simulink model "Drive_DC"  (R2022b)
settings: Solver=VariableStepAuto  StartTime=0.0  StopTime=13  MaxStep=1e-5  RelTol=1e-3
undefined symbols (not defined in the file or in its folder): DiscIntNeverNeededParam, sigbuilder_block
libraries: spsMeanLib x6, slpidlib x5, simulink_extras x5, spsSawtoothGeneratorLib x4, simulink x2, pid_lib x1, spspowerguiLib x1
(part 1 of 2)
settings Model: Creator=AHMED  LastModifiedBy=moham
settings SolverCC: ZeroCrossAlgorithm=Adaptive
settings DebuggingCC: MaskedZcDiagnostic=none  IgnoredZcDiagnostic=none  UnconnectedInputMsg=warning  UnconnectedOutputMsg=warning  UnconnectedLineMsg=warning
settings ModelReferenceCC: EnableRefExpFcnMdlSchedulingChecks=on
settings RTWCC: DLArmComputeVersion=19.05

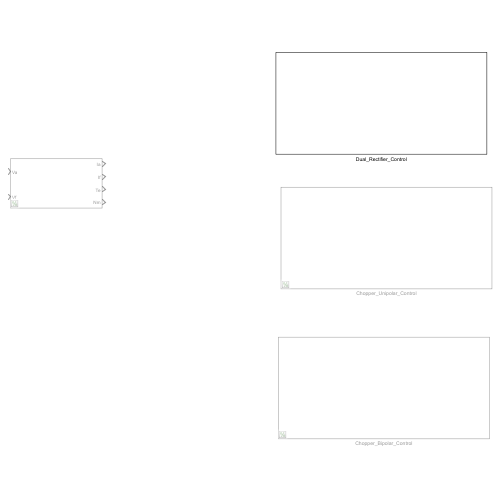
[thumbnail: Simulink's stored preview of the top-level diagram]
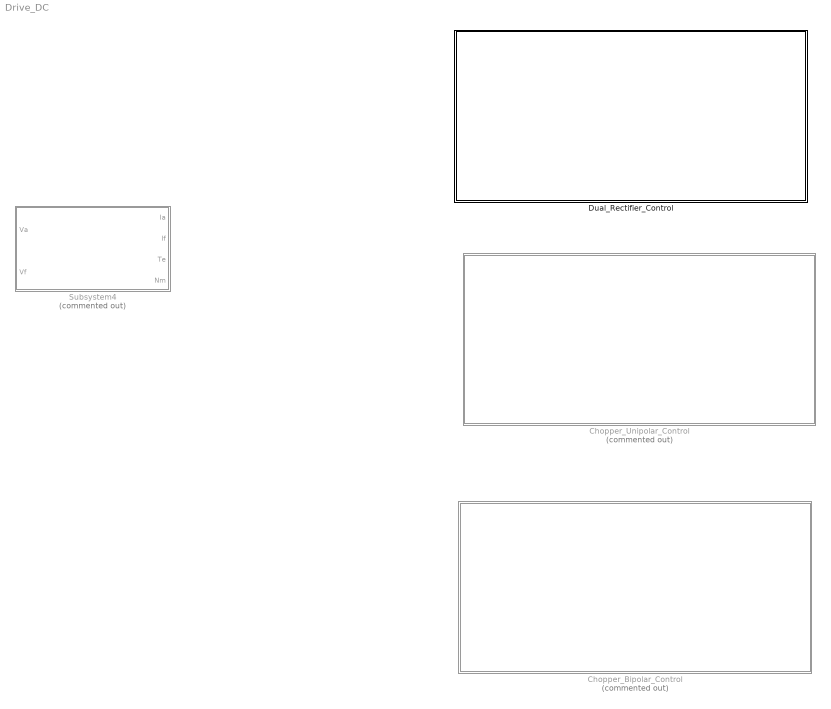
== system Drive_DC ==
  Chopper_Bipolar_Control : Subsystem  Commented=on
  Chopper_Unipolar_Control : Subsystem  Commented=on
  Dual_Rectifier_Control : Subsystem
  Subsystem4 : Subsystem  Commented=on  mask{Ra=0.6, Rf=240, La=12e-3, Lf=120, J=0.1, k=1.309}

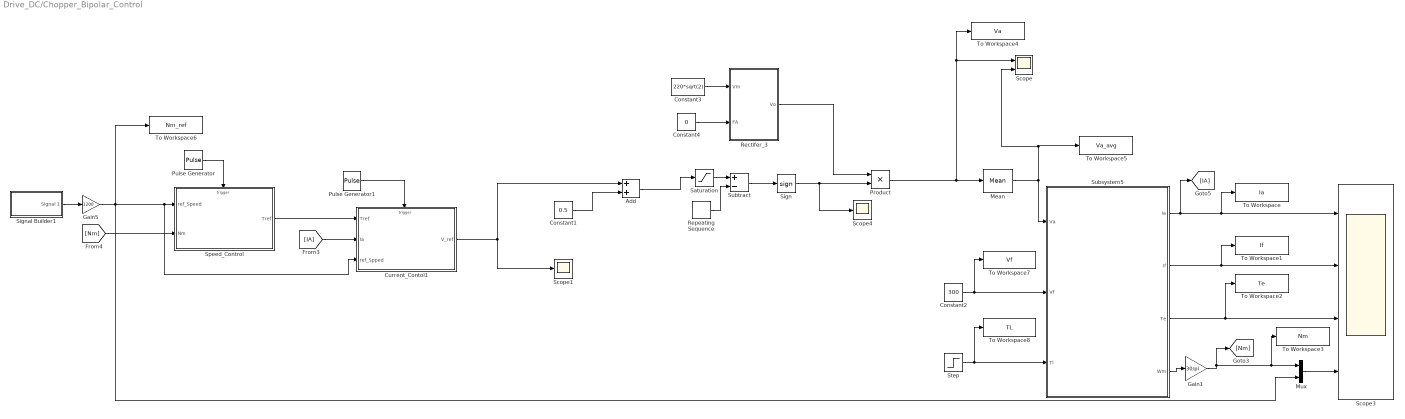
== system Drive_DC/Chopper_Bipolar_Control ==
  Add : Sum
  Constant1 : Constant  Value=0.5
  Constant2 : Constant  Value=300
  Constant3 : Constant  Value=220*sqrt(2)
  Constant4 : Constant  Value=0
  Current_Contol1 : Subsystem
  Gain1 : Gain  Gain=30/pi
  Gain5 : Gain  Gain=1200
  Mean : spsMeanLib/Mean  Freq=50  Vinit=0  Ts=0
  Mux : Mux  Inputs=2
  Product : Product
  Pulse Generator : DiscretePulseGenerator  PulseType=Time based  Period=1/1000  PulseWidth=50
  Pulse Generator1 : DiscretePulseGenerator  PulseType=Time based  Period=1/10000  PulseWidth=50
  Rectifer_3 : Subsystem
  Repeating Sequence : simulink/Sources/Repeating Sequence  rep_seq_t=[0 0.5/10000 1/10000]  rep_seq_y=[0 1 0]
  Saturation : Saturate  UpperLimit=1  LowerLimit=0
  Scope : Scope  NumInputPorts=2
  Scope1 : Scope
  Scope3 : Scope  NumInputPorts=4
  Scope4 : Scope
  Sign : Signum
  Signal Builder1 : Subsystem  Tag=STV Subsys  LoadFcn=sigbuilder_block('load');  StartFcn=sigbuilder_block('start');  StopFcn=sigbuilder_block('stop');  ClipboardFcn=sigbuilder_block('clipboard');  mask(Sigbuilder block){tuvar=[0:10]}
      mask help: Simulink:masks:SigbuilderBlock_MD
      mask init:
      | if ~strcmp(get_param(bdroot(gcbh),'SimulationStatus'),'stopped') tuvar = sigbuilder_block('maskInit'); end
      settings: CopyFcn=sigbuilder_block('copy');  DeleteFcn=sigbuilder_block('delete');  ModelCloseFcn=sigbuilder_block('modelClose');  PreSaveFcn=sigbuilder_block('preSave');  PauseFcn=sigbuilder_block('pause');  ContinueFcn=sigbuilder_block('continue');  NameChangeFcn=sigbuilder_block('namechange');  OpenFcn=sigbuilder_block('open',[5.4 30 1141.2 522.6 ]);  CloseFcn=sigbuilder_block('close');
      mask Display: plot(0, 0, 100, 100,[2, 2, 32, 32, 2], [68, 8, 8, 68, 68],[32, 2], [38, 38], [32, 19, 2],[53, 60, 44], [32, 17, 17, 2],[16, 16, 31, 31]);txt = getActiveGroup(gcbh);text(2, 100, txt,'verticalAlignment', 'top');
  Speed_Control : Subsystem
  Step : Step  Time=2.25  After=5  SampleTime=0
  Subsystem5 : Subsystem  mask{Ra=0.6, Rf=240, La=12e-3, Lf=120, J=0.05, k=1.309}
  Subtract : Sum  Inputs=+-
  To Workspace : ToWorkspace  VariableName=Ia  SaveFormat=Structure With Time  SampleTime=-1
  To Workspace1 : ToWorkspace  VariableName=If  SaveFormat=Structure With Time  SampleTime=-1
  To Workspace2 : ToWorkspace  VariableName=Te  SaveFormat=Structure With Time  SampleTime=-1
  To Workspace3 : ToWorkspace  VariableName=Nm  SaveFormat=Structure With Time  SampleTime=-1
  To Workspace4 : ToWorkspace  VariableName=Va  SaveFormat=Structure With Time  SampleTime=-1
  To Workspace5 : ToWorkspace  VariableName=Va_avg  SaveFormat=Structure With Time  SampleTime=-1
  To Workspace6 : ToWorkspace  VariableName=Nm_ref  SaveFormat=Structure With Time  SampleTime=-1
  To Workspace7 : ToWorkspace  VariableName=Vf  SaveFormat=Structure With Time  SampleTime=-1
  To Workspace8 : ToWorkspace  VariableName=TL  SaveFormat=Structure With Time  SampleTime=-1
  wires:
  Subtract/1 -> Sign/1
  Mean/1 -> Subsystem5/1(Va), To Workspace5/1, Scope/2
  Rectifer_3/1(Vo) -> Product/1
  Sign/1 -> Scope4/1, Product/2
  Current_Contol1/1(V_ref) -> Add/1, Scope1/1
  Repeating Sequence/1 -> Subtract/2
  Gain1/1 -> Mux/1, To Workspace3/1, [Nm]
  Subsystem5/2(If) -> Scope3/2, To Workspace1/1
  Mux/1 -> Scope3/4
  Step/1 -> To Workspace8/1, Subsystem5/3(Tl)
  Speed_Control/1(Tref) -> Current_Contol1/1(Tref)
  Constant2/1 -> To Workspace7/1, Subsystem5/2(Vf)
  Product/1 -> To Workspace4/1, Scope/1, Mean/1
  [IA] -> Current_Contol1/2(Ia)
  Subsystem5/4(Wm) -> Gain1/1
  Signal Builder1/1(Signal 1) -> Gain5/1
  Gain5/1 -> To Workspace6/1, Mux/2, Current_Contol1/3("ref_Spped "), Speed_Control/1(ref_Speed)
  [Nm] -> Speed_Control/2("Nm ")
  Pulse Generator/1 -> Speed_Control/Trigger
  Subsystem5/3(Te) -> Scope3/3, To Workspace2/1
  Pulse Generator1/1 -> Current_Contol1/Trigger
  Subsystem5/1(Ia) -> [IA], Scope3/1, To Workspace/1
  Constant1/1 -> Add/2
  Add/1 -> Saturation/1
  Saturation/1 -> Subtract/1
  Constant3/1 -> Rectifer_3/1(Vm)
  Constant4/1 -> Rectifer_3/2(FA)

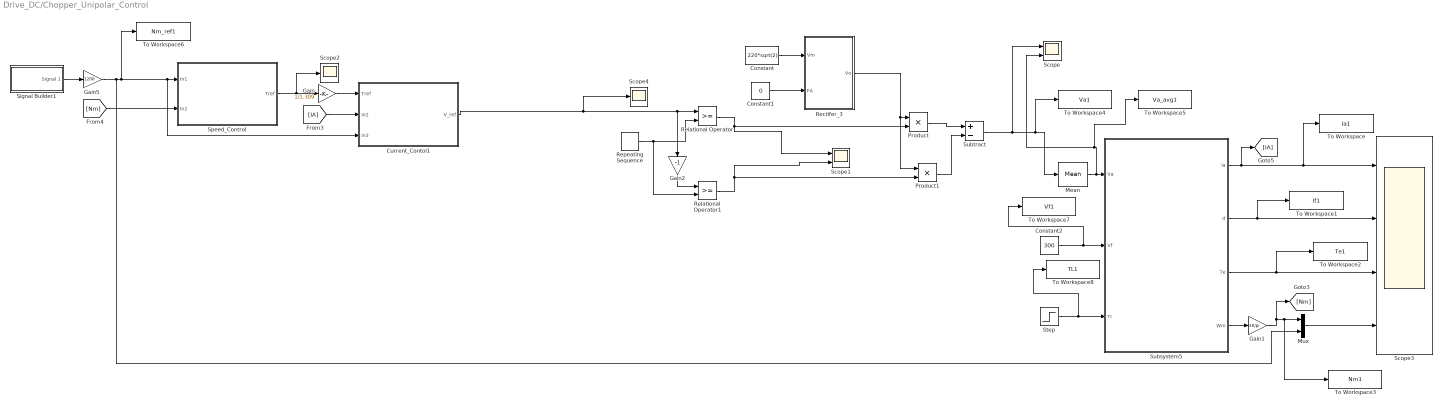
== system Drive_DC/Chopper_Unipolar_Control ==
  Constant : Constant  Value=220*sqrt(2)
  Constant1 : Constant  Value=0
  Constant2 : Constant  Value=300
  Current_Contol1 : Subsystem
  Gain : Gain  Gain=1/1.309
  Gain1 : Gain  Gain=30/pi
  Gain2 : Gain  Gain=-1
  Gain5 : Gain  Gain=1200
  Mean : spsMeanLib/Mean  Freq=50  Vinit=0  Ts=0
  Mux : Mux  Inputs=2
  Product : Product
  Product1 : Product
  Rectifer_3 : Subsystem
  Relational Operator : RelationalOperator  OutDataTypeStr=boolean  RndMeth=Simplest  InputSameDT=off
  Relational Operator1 : RelationalOperator  OutDataTypeStr=boolean  RndMeth=Simplest  InputSameDT=off
  Repeating Sequence : simulink/Sources/Repeating Sequence  rep_seq_t=[0 0.5/1000 1/1000]  rep_seq_y=[0 1 0]
  Scope : Scope  NumInputPorts=2
  Scope1 : Scope  NumInputPorts=2
  Scope2 : Scope
  Scope3 : Scope  NumInputPorts=4
  Scope4 : Scope
  Signal Builder1 : Subsystem  Tag=STV Subsys  LoadFcn=sigbuilder_block('load');  StartFcn=sigbuilder_block('start');  StopFcn=sigbuilder_block('stop');  ClipboardFcn=sigbuilder_block('clipboard');  mask(Sigbuilder block){tuvar=[0:10]}
      mask help: Simulink:masks:SigbuilderBlock_MD
      mask init:
      | if ~strcmp(get_param(bdroot(gcbh),'SimulationStatus'),'stopped') tuvar = sigbuilder_block('maskInit'); end
      settings: CopyFcn=sigbuilder_block('copy');  DeleteFcn=sigbuilder_block('delete');  ModelCloseFcn=sigbuilder_block('modelClose');  PreSaveFcn=sigbuilder_block('preSave');  PauseFcn=sigbuilder_block('pause');  ContinueFcn=sigbuilder_block('continue');  NameChangeFcn=sigbuilder_block('namechange');  OpenFcn=sigbuilder_block('open',[5.4 30 1141.2 522.6 ]);  CloseFcn=sigbuilder_block('close');
      mask Display: plot(0, 0, 100, 100,[2, 2, 32, 32, 2], [68, 8, 8, 68, 68],[32, 2], [38, 38], [32, 19, 2],[53, 60, 44], [32, 17, 17, 2],[16, 16, 31, 31]);txt = getActiveGroup(gcbh);text(2, 100, txt,'verticalAlignment', 'top');
  Speed_Control : Subsystem
  Step : Step  Time=2.25  After=5  SampleTime=0
  Subsystem5 : Subsystem  mask{Ra=0.6, Rf=240, La=12e-3, Lf=120, J=0.05, k=1.309}
  Subtract : Sum  Inputs=+-
  To Workspace : ToWorkspace  VariableName=Ia1  SaveFormat=Structure With Time  SampleTime=-1
  To Workspace1 : ToWorkspace  VariableName=If1  SaveFormat=Structure With Time  SampleTime=-1
  To Workspace2 : ToWorkspace  VariableName=Te1  SaveFormat=Structure With Time  SampleTime=-1
  To Workspace3 : ToWorkspace  VariableName=Nm1  SaveFormat=Structure With Time  SampleTime=-1
  To Workspace4 : ToWorkspace  VariableName=Va1  SaveFormat=Structure With Time  SampleTime=-1
  To Workspace5 : ToWorkspace  VariableName=Va_avg1  SaveFormat=Structure With Time  SampleTime=-1
  To Workspace6 : ToWorkspace  VariableName=Nm_ref1  SaveFormat=Structure With Time  SampleTime=-1
  To Workspace7 : ToWorkspace  VariableName=Vf1  SaveFormat=Structure With Time  SampleTime=-1
  To Workspace8 : ToWorkspace  VariableName=TL1  SaveFormat=Structure With Time  SampleTime=-1
  wires:
  Subsystem5/3(Te) -> To Workspace2/1, Scope3/3
  [Nm] -> Speed_Control/2(In2)
  Gain5/1 -> To Workspace6/1, Speed_Control/1(In1), Current_Contol1/3(In3), Mux/2
  Signal Builder1/1(Signal 1) -> Gain5/1
  Subsystem5/4(Wm) -> Gain1/1
  [IA] -> Current_Contol1/2(In2)
  Subtract/1 -> Scope/1, To Workspace4/1, Mean/1
  Constant2/1 -> To Workspace7/1, Subsystem5/2(Vf)
  Speed_Control/1(Tref) -> Scope2/1, Gain/1
  Step/1 -> To Workspace8/1, Subsystem5/3(Tl)
  Mux/1 -> Scope3/4
  Subsystem5/1(Ia) -> To Workspace/1, Scope3/1, [IA]
  Subsystem5/2(If) -> To Workspace1/1, Scope3/2
  Gain1/1 -> [Nm], To Workspace3/1, Mux/1
  Repeating Sequence/1 -> Relational Operator1/2, Relational Operator/2
  Current_Contol1/1(V_ref) -> Scope4/1, Relational Operator/1, Gain2/1
  Rectifer_3/1(Vo) -> Product1/1, Product/1
  Product/1 -> Subtract/1
  Product1/1 -> Subtract/2
  Mean/1 -> To Workspace5/1, Scope/2, Subsystem5/1(Va)
  Relational Operator/1 -> Product/2, Scope1/1
  Relational Operator1/1 -> Product1/2, Scope1/2
  Gain2/1 -> Relational Operator1/1
  Constant/1 -> Rectifer_3/1(Vm)
  Constant1/1 -> Rectifer_3/2(FA)
  Gain/1 -> Current_Contol1/1(Tref)

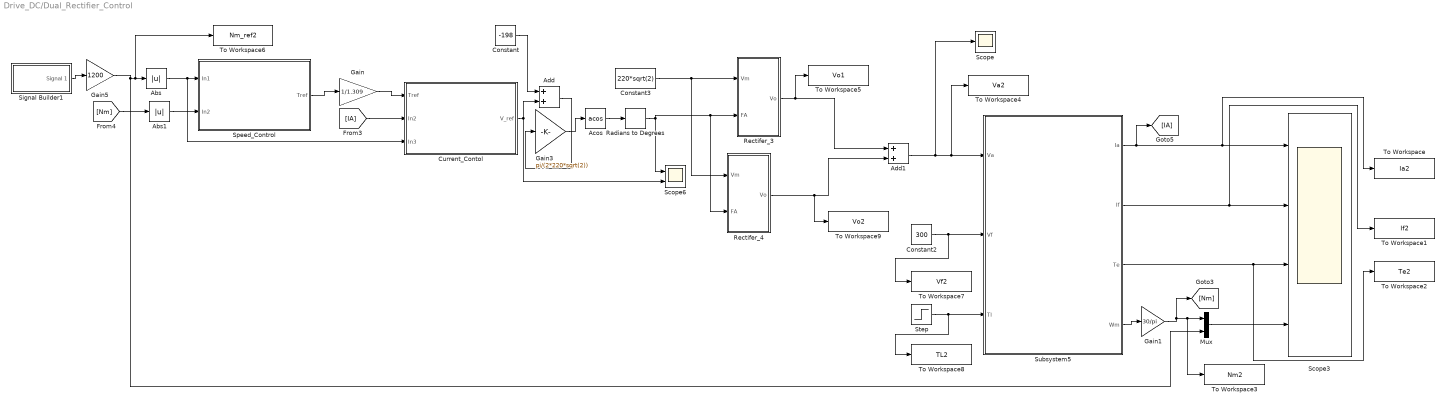
== system Drive_DC/Dual_Rectifier_Control ==
  Abs : Abs  SaturateOnIntegerOverflow=off
  Abs1 : Abs  SaturateOnIntegerOverflow=off
  Acos : Trigonometry  Operator=acos
  Add : Sum
  Add1 : Sum
  Constant : Constant  Value=-198
  Constant2 : Constant  Value=300
  Constant3 : Constant  Value=220*sqrt(2)
  Current_Contol : Subsystem
  Gain : Gain  Gain=1/1.309
  Gain1 : Gain  Gain=30/pi
  Gain3 : Gain  Gain=pi/(2*220*sqrt(2))
  Gain5 : Gain  Gain=1200
  Mux : Mux  Inputs=2
  Radians to Degrees : simulink_extras/Transformations/Radians to Degrees
  Rectifer_3 : Subsystem
  Rectifer_4 : Subsystem
  Scope : Scope
  Scope3 : Scope  NumInputPorts=4
  Scope6 : Scope  NumInputPorts=2
  Signal Builder1 : Subsystem  Tag=STV Subsys  LoadFcn=sigbuilder_block('load');  StartFcn=sigbuilder_block('start');  StopFcn=sigbuilder_block('stop');  ClipboardFcn=sigbuilder_block('clipboard');  mask(Sigbuilder block){tuvar=[0:10]}
      mask help: Simulink:masks:SigbuilderBlock_MD
      mask init:
      | if ~strcmp(get_param(bdroot(gcbh),'SimulationStatus'),'stopped') tuvar = sigbuilder_block('maskInit'); end
      settings: CopyFcn=sigbuilder_block('copy');  DeleteFcn=sigbuilder_block('delete');  ModelCloseFcn=sigbuilder_block('modelClose');  PreSaveFcn=sigbuilder_block('preSave');  PauseFcn=sigbuilder_block('pause');  ContinueFcn=sigbuilder_block('continue');  NameChangeFcn=sigbuilder_block('namechange');  OpenFcn=sigbuilder_block('open',[5.4 30 1141.2 522.6 ]);  CloseFcn=sigbuilder_block('close');
      mask Display: plot(0, 0, 100, 100,[2, 2, 32, 32, 2], [68, 8, 8, 68, 68],[32, 2], [38, 38], [32, 19, 2],[53, 60, 44], [32, 17, 17, 2],[16, 16, 31, 31]);txt = getActiveGroup(gcbh);text(2, 100, txt,'verticalAlignment', 'top');
  Speed_Control : Subsystem
  Step : Step  Time=2.25  After=5  SampleTime=0
  Subsystem5 : Subsystem  mask{Ra=0.6, Rf=240, La=12e-3, Lf=120, J=0.05, k=1.309}
  To Workspace : ToWorkspace  VariableName=Ia2  SaveFormat=Structure With Time  SampleTime=-1
  To Workspace1 : ToWorkspace  VariableName=If2  SaveFormat=Structure With Time  SampleTime=-1
  To Workspace2 : ToWorkspace  VariableName=Te2  SaveFormat=Structure With Time  SampleTime=-1
  To Workspace3 : ToWorkspace  VariableName=Nm2  SaveFormat=Structure With Time  SampleTime=-1
  To Workspace4 : ToWorkspace  VariableName=Va2  SaveFormat=Structure With Time  SampleTime=-1
  To Workspace5 : ToWorkspace  VariableName=Vo1  SaveFormat=Structure With Time  SampleTime=-1
  To Workspace6 : ToWorkspace  VariableName=Nm_ref2  SaveFormat=Structure With Time  SampleTime=-1
  To Workspace7 : ToWorkspace  VariableName=Vf2  SaveFormat=Structure With Time  SampleTime=-1
  To Workspace8 : ToWorkspace  VariableName=TL2  SaveFormat=Structure With Time  SampleTime=-1
  To Workspace9 : ToWorkspace  VariableName=Vo2  SaveFormat=Structure With Time  SampleTime=-1
  wires:
  [Nm] -> Abs1/1
  Gain1/1 -> To Workspace3/1, Mux/1, [Nm]
  Gain5/1 -> Mux/2, To Workspace6/1, Abs/1
  Subsystem5/2(If) -> To Workspace1/1, Scope3/2
  Subsystem5/1(Ia) -> [IA], To Workspace/1, Scope3/1
  Mux/1 -> Scope3/4
  Step/1 -> To Workspace8/1, Subsystem5/3(Tl)
  Gain3/1 -> Acos/1
  Speed_Control/1(Tref) -> Gain/1
  Constant2/1 -> To Workspace7/1, Subsystem5/2(Vf)
  Acos/1 -> Radians to Degrees/1
  Add1/1 -> Scope/1, To Workspace4/1, Subsystem5/1(Va)
  Radians to Degrees/1 -> Rectifer_4/2(FA), Rectifer_3/2(FA), Scope6/1
  [IA] -> Current_Contol/2(In2)
  Subsystem5/4(Wm) -> Gain1/1
  Signal Builder1/1(Signal 1) -> Gain5/1
  Abs/1 -> Current_Contol/3(In3), Speed_Control/1(In1)
  Abs1/1 -> Speed_Control/2(In2)
  Constant3/1 -> Rectifer_3/1(Vm), Rectifer_4/1(Vm)
  Current_Contol/1(V_ref) -> Add/2, Scope6/2
  Subsystem5/3(Te) -> To Workspace2/1, Scope3/3
  Add/1 -> Gain3/1
  Constant/1 -> Add/1
  Gain/1 -> Current_Contol/1(Tref)
  Rectifer_3/1(Vo) -> To Workspace5/1, Add1/1
  Rectifer_4/1(Vo) -> To Workspace9/1, Add1/2

== system Drive_DC/Subsystem4 ==
  Va : Inport
  Vf : Inport  Port=2
  Constant : Constant  Value=1000
  Gain : Gain  Gain=pi/30
  Subsystem : Subsystem
  Subsystem1 : Subsystem
  Subsystem3 : Subsystem
  Ia : Outport
  If : Outport  Port=2
  Te : Outport  Port=3
  Nm : Outport  Port=4
  wires:
  Va/1 -> Subsystem/1(Va)
  Subsystem/1(Ia) -> Subsystem1/1(Ia), Ia/1
  Subsystem1/1(Te) -> Te/1
  Vf/1 -> Subsystem3/1(In1)
  Subsystem3/1(Out1) -> If/1
  Constant/1 -> Gain/1
  Gain/1 -> Nm/1, Subsystem/2(W)

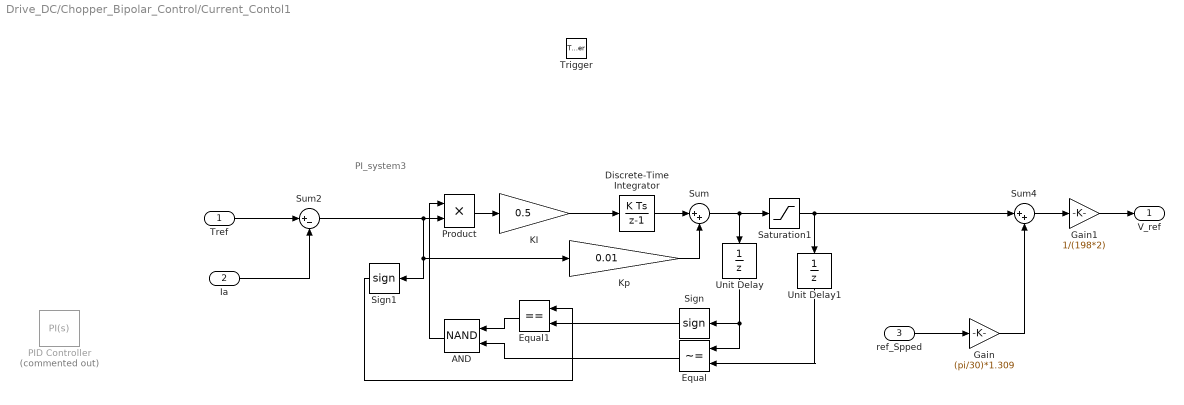
== system Drive_DC/Chopper_Bipolar_Control/Current_Contol1 ==
  note: PI_system3
  Tref : Inport
  Ia : Inport  Port=2
  "ref_Spped " : Inport  Port=3
  Trigger : TriggerPort  VariantControl=(inherit)  PortDimensions=1
  AND : Logic  Operator=NAND  AllPortsSameDT=off  OutDataTypeStr=boolean
  Discrete-Time Integrator : DiscreteIntegrator  SampleTime=-1  ICPrevOutput=DiscIntNeverNeededParam  ICPrevScaledInput=DiscIntNeverNeededParam
  Equal : RelationalOperator  Operator=~=  OutDataTypeStr=boolean  RndMeth=Simplest  InputSameDT=off
  Equal1 : RelationalOperator  Operator===  OutDataTypeStr=boolean  RndMeth=Simplest  InputSameDT=off
  Gain : Gain  Gain=(pi/30)*1.309
  Gain1 : Gain  Gain=1/(198*2)
  KI : Gain  Gain=0.5
  Kp : Gain  Gain=0.01
  PID Controller : slpidlib/PID Controller  Commented=on  Controller=PI  Form=Parallel  TimeDomain=Continuous-time  UseExternalTs=off  SampleTime=-1  IntegratorMethod=Forward Euler  FilterMethod=Forward Euler  ControllerParametersSource=internal  P=0.1  I=10  UseKiTs=off  D=0  N=100  UseFilter=on  TunerSelectOption=Transfer Function Based (PID Tuner App)  InitialConditionSource=internal  InitialConditionForIntegrator=0  InitialConditionForFilter=0  DifferentiatorICPrevScaledInput=0  ExternalReset=none  TrackingMode=off  Kt=1  LimitOutput=on  SatLimitsSource=internal  UpperSaturationLimit=240  LowerSaturationLimit=-240  LinearizeAsGain=on  AntiWindupMode=clamping  Kb=1  LimitIntegrator=off  UpperIntegratorSaturationLimit=inf  LowerIntegratorSaturationLimit=-inf  POutMin=[]  POutMax=[]  IOutMin=[]  IOutMax=[]  DOutMin=[]  DOutMax=[]  NOutMin=[]  NOutMax=[]  SumOutMin=[]  SumOutMax=[]  SaturationOutMin=[]  SaturationOutMax=[]  PParamMin=[]  PParamMax=[]  IParamMin=[]  IParamMax=[]  DParamMin=[]  DParamMax=[]  NParamMin=[]  NParamMax=[]  KbParamMin=[]  KbParamMax=[]  KtParamMin=[]  KtParamMax=[]  KbOutMin=[]  KbOutMax=[]  KtOutMin=[]  KtOutMax=[]  IntegratorOutMin=[]  IntegratorOutMax=[]  FilterOutMin=[]  FilterOutMax=[]  SumI1OutMin=[]  SumI1OutMax=[]  SumI2OutMin=[]  SumI2OutMax=[]  SumI3OutMin=[]  SumI3OutMax=[]  SumI4OutMin=[]  SumI4OutMax=[]  SumDOutMin=[]  SumDOutMax=[]  DifferentiatorOutMin=[]  DifferentiatorOutMax=[]  FilterDiffOutCoefMin=[]  FilterDiffOutCoefMax=[]  ReciprocalOutMin=[]  ReciprocalOutMax=[]  SumDenOutMin=[]  SumDenOutMax=[]  SumNumOutMin=[]  SumNumOutMax=[]  DivideOutMin=[]  DivideOutMax=[]  UdiffTsProdOutMin=[]  UdiffTsProdOutMax=[]  NTsProdOutMin=[]  NTsProdOutMax=[]  UintegralTsProdOutMin=[]  UintegralTsProdOutMax=[]  UngainTsProdOutMin=[]  UngainTsProdOutMax=[]  ClampingZeroOutDataTypeStr=Inherit: Inherit via back propagation  ClampingZeroOutMin=[]  ClampingZeroOutMax=[]  FilterDenConstantOutDataTypeStr=Inherit: Inherit via back propagation  FilterDenConstantOutMin=[]  FilterDenConstantOutMax=[]  PCopyOutDataTypeStr=Inherit: Inherit via back propagation  PCopyOutMin=[]  PCopyOutMax=[]  NCopyOutDataTypeStr=Inherit: Inherit via back propagation  NCopyOutMin=[]  NCopyOutMax=[]  IntegratorContinuousStateAttributes=''  IntegratorStateMustResolveToSignalObject=off  IntegratorRTWStateStorageClass=Auto  FilterContinuousStateAttributes=''  FilterStateMustResolveToSignalObject=off  FilterRTWStateStorageClass=Auto  ParallelPVariant=InternalParameters  IdealPVariant=Disabled  IVariant=InternalParameters  DVariant=Disabled  IntegratorVariant=Continuous  SatVariant=Enabled  AWVariant=ContClampingParallel  PCopyVariant=Disabled  TRVariant=Disabled  FdbkBlocksVariant=Forward  IdealPFdbkVariant=Disabled  SatFdbkVariant=Disabled  DerivativeFilterVariant=Disabled  NVariant=Disabled  NCopyVariant=Disabled_SignalSpec  FilterICVariant=Disabled  IntegratorICVariant=InternalICs  ExternalResetVariant=Disabled  TRSumVariant=Passthrough  SumFdbkVariant=Disabled  SumVariant=Sum_PI  TsampFilterVariant=InternalTs  TsampNgainVariant=Passthrough  TsampIntegralVariant=Passthrough  ExternalSaturationOutDataTypeStr=Inherit: Same as second input
  Product : Product
  Saturation1 : Saturate  UpperLimit=198*2  LowerLimit=0
  Sign : Signum
  Sign1 : Signum
  Sum : Sum  Inputs=|++
  Sum2 : Sum  Inputs=|+-
  Sum4 : Sum  Inputs=|++
  Unit Delay : UnitDelay  SampleTime=-1  HasFrameUpgradeWarning=on
  Unit Delay1 : UnitDelay  SampleTime=-1  HasFrameUpgradeWarning=on
  V_ref : Outport
  wires:
  Gain1/1 -> V_ref/1
  Tref/1 -> Sum2/1
  Ia/1 -> Sum2/2
  "ref_Spped "/1 -> Gain/1
  Gain/1 -> Sum4/2
  Discrete-Time Integrator/1 -> Sum/1
  Kp/1 -> Sum/2
  KI/1 -> Discrete-Time Integrator/1
  Sum/1 -> Saturation1/1, Unit Delay/1
  Saturation1/1 -> Sum4/1, Unit Delay1/1
  Sign/1 -> Equal1/2
  Sign1/1 -> Equal1/1
  Equal1/1 -> AND/1
  Equal/1 -> AND/2
  Unit Delay/1 -> Equal/1, Sign/1
  Product/1 -> KI/1
  Unit Delay1/1 -> Equal/2
  AND/1 -> Product/1
  Sum2/1 -> Kp/1, Sign1/1, Product/2
  Sum4/1 -> Gain1/1

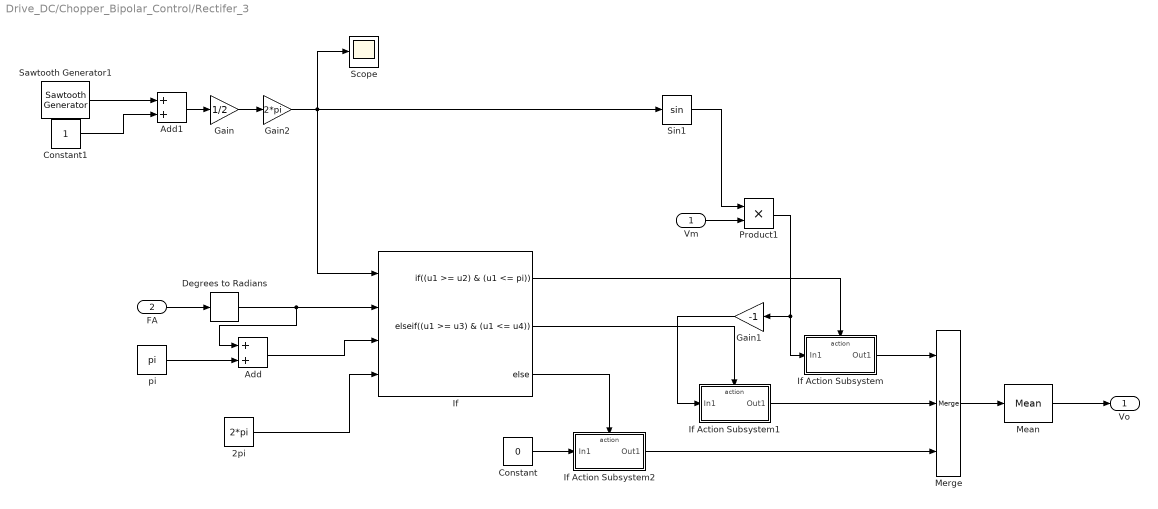
== system Drive_DC/Chopper_Bipolar_Control/Rectifer_3 ==
  Vm : Inport
  FA : Inport  Port=2
  2pi : Constant  Value=2*pi
  Add : Sum
  Add1 : Sum
  Constant : Constant  Value=0
  Constant1 : Constant
  Degrees to Radians : simulink_extras/Transformations/Degrees to Radians
  Gain : Gain  Gain=1/2
  Gain1 : Gain  Gain=-1
  Gain2 : Gain  Gain=2*pi
  If : If  NumInputs=4  IfExpression=(u1 >= u2) & (u1 <= pi)  ElseIfExpressions=(u1 >= u3) & (u1 <= u4)
  If Action Subsystem : Subsystem  TreatAsAtomicUnit=on
  If Action Subsystem1 : Subsystem  TreatAsAtomicUnit=on
  If Action Subsystem2 : Subsystem  TreatAsAtomicUnit=on
  Mean : spsMeanLib/Mean  Freq=50  Vinit=0  Ts=0
  Merge : Merge  Inputs=3
  Product1 : Product
  Sawtooth Generator1 : spsSawtoothGeneratorLib/Sawtooth Generator  Freq=50  Phase=180  Ts=0
  Scope : Scope
  Sin1 : Trigonometry
  pi : Constant  Value=pi
  Vo : Outport
  wires:
  Gain2/1 -> Sin1/1, If/1, Scope/1
  Gain/1 -> Gain2/1
  Add1/1 -> Gain/1
  Constant1/1 -> Add1/2
  Sawtooth Generator1/1 -> Add1/1
  Constant/1 -> If Action Subsystem2/1(In1)
  Gain1/1 -> If Action Subsystem1/1(In1)
  Product1/1 -> Gain1/1, If Action Subsystem/1(In1)
  Sin1/1 -> Product1/1
  Merge/1 -> Mean/1
  If Action Subsystem2/1(Out1) -> Merge/3
  If Action Subsystem1/1(Out1) -> Merge/2
  If Action Subsystem/1(Out1) -> Merge/1
  If/3 -> If Action Subsystem2/Action
  If/2 -> If Action Subsystem1/Action
  If/1 -> If Action Subsystem/Action
  2pi/1 -> If/4
  Add/1 -> If/3
  pi/1 -> Add/2
  Degrees to Radians/1 -> If/2, Add/1
  FA/1 -> Degrees to Radians/1
  Mean/1 -> Vo/1
  Vm/1 -> Product1/2

== system Drive_DC/Chopper_Bipolar_Control/Signal Builder1 ==
  Demux : Demux  Tag=STV Demux  Outputs=1
      settings: DisplayOption=none
  FromWs : FromWorkspace  Tag=STV FromWs  VariableName=tuvar
      SigBuilderData=|
      | common.afterFinalStr = 'Extrapolate'
      | common.sampleTime = 0
      | dataSet.timeRange = [0 13]
      | dataSet.name = 'Group 1'
      | sbobj.Groups.Name = 'Group 1'
      | sbobj.Groups.Signals.Name = 'Signal 1'
      | sbobj.Groups.Signals.XData = [0 1 2 3 4 5 8 9 10 11 12 13]
      | sbobj.Groups.Signals.YData = [0 0 0.5 0.5 1 1 -0.5 -0.5 -0.85 -0.85 -0.01 -0.01]
      | sbobj.Groups.TimeRange = [0 13]
  Signal 1 : Outport  Tag=STV Outport
  wires:
  Demux/1 -> Signal 1/1
  FromWs/1 -> Demux/1

== system Drive_DC/Chopper_Bipolar_Control/Speed_Control ==
  note: PI_system3
  ref_Speed : Inport
  "Nm " : Inport  Port=2
  Trigger : TriggerPort  VariantControl=(inherit)  PortDimensions=1
  AND : Logic  Operator=NAND  AllPortsSameDT=off  OutDataTypeStr=boolean
  Discrete-Time Integrator : DiscreteIntegrator  SampleTime=-1  ICPrevOutput=DiscIntNeverNeededParam  ICPrevScaledInput=DiscIntNeverNeededParam
  Equal : RelationalOperator  Operator=~=  OutDataTypeStr=boolean  RndMeth=Simplest  InputSameDT=off
  Equal1 : RelationalOperator  Operator===  OutDataTypeStr=boolean  RndMeth=Simplest  InputSameDT=off
  KI : Gain  Gain=0.7
  Kp : Gain  Gain=0.5
  PID Controller : pid_lib/PID Controller  Commented=on  Controller=PI  Form=Parallel  TimeDomain=Continuous-time  UseExternalTs=off  SampleTime=-1  IntegratorMethod=Forward Euler  FilterMethod=Forward Euler  ControllerParametersSource=internal  P=0.5  I=0.5  D=0  UseFilter=on  N=100  TunerSelectOption=Transfer Function Based (PID Tuner App)  InitialConditionSource=internal  InitialConditionForIntegrator=0  InitialConditionForFilter=0  DifferentiatorICPrevScaledInput=0  ExternalReset=none  TrackingMode=off  Kt=1  LimitOutput=on  SatLimitsSource=internal  UpperSaturationLimit=(30*746)/(1740*pi/30)  LowerSaturationLimit=-(30*746)/(1740*pi/30)  LinearizeAsGain=on  AntiWindupMode=clamping  Kb=1  POutMin=[]  POutMax=[]  IOutMin=[]  IOutMax=[]  DOutMin=[]  DOutMax=[]  NOutMin=[]  NOutMax=[]  SumOutMin=[]  SumOutMax=[]  SaturationOutMin=[]  SaturationOutMax=[]  PParamMin=[]  PParamMax=[]  IParamMin=[]  IParamMax=[]  DParamMin=[]  DParamMax=[]  NParamMin=[]  NParamMax=[]  KbParamMin=[]  KbParamMax=[]  KtParamMin=[]  KtParamMax=[]  KbOutMin=[]  KbOutMax=[]  KtOutMin=[]  KtOutMax=[]  IntegratorOutMin=[]  IntegratorOutMax=[]  FilterOutMin=[]  FilterOutMax=[]  SumI1OutMin=[]  SumI1OutMax=[]  SumI2OutMin=[]  SumI2OutMax=[]  SumI3OutMin=[]  SumI3OutMax=[]  SumI4OutMin=[]  SumI4OutMax=[]  SumDOutMin=[]  SumDOutMax=[]  DifferentiatorOutMin=[]  DifferentiatorOutMax=[]  FilterDiffOutCoefMin=[]  FilterDiffOutCoefMax=[]  ReciprocalOutMin=[]  ReciprocalOutMax=[]  SumDenOutMin=[]  SumDenOutMax=[]  SumNumOutMin=[]  SumNumOutMax=[]  DivideOutMin=[]  DivideOutMax=[]  UdiffTsProdOutMin=[]  UdiffTsProdOutMax=[]  NTsProdOutMin=[]  NTsProdOutMax=[]  UintegralTsProdOutMin=[]  UintegralTsProdOutMax=[]  UngainTsProdOutMin=[]  UngainTsProdOutMax=[]  IntegratorContinuousStateAttributes=''  IntegratorStateMustResolveToSignalObject=off  IntegratorRTWStateStorageClass=Auto  FilterContinuousStateAttributes=''  FilterStateMustResolveToSignalObject=off  FilterRTWStateStorageClass=Auto  ParallelPVariant=InternalParameters  IdealPVariant=Disabled  IVariant=InternalParameters  DVariant=Disabled  IntegratorVariant=Continuous  SatVariant=Enabled  AWVariant=ContClampingParallel  PCopyVariant=Disabled  TRVariant=Disabled  FdbkBlocksVariant=Forward  IdealPFdbkVariant=Disabled  SatFdbkVariant=Disabled  DerivativeFilterVariant=Disabled  NVariant=Disabled  NCopyVariant=Disabled_SignalSpec  FilterICVariant=Disabled  IntegratorICVariant=InternalICs  ExternalResetVariant=Disabled  TRSumVariant=Passthrough  SumFdbkVariant=Disabled  SumVariant=Sum_PI  TsampFilterVariant=InternalTs  TsampNgainVariant=Passthrough  TsampIntegralVariant=Passthrough  ExternalSaturationOutDataTypeStr=Inherit: Same as second input
  Product : Product
  Saturation2 : Saturate  UpperLimit=(30*746)/(1740*pi/30)  LowerLimit=-(30*746)/(1740*pi/30)
  Sign : Signum
  Sign1 : Signum
  Sum : Sum  Inputs=|+-
  Sum2 : Sum  Inputs=|++
  Unit Delay : UnitDelay  SampleTime=-1  HasFrameUpgradeWarning=on
  Unit Delay1 : UnitDelay  SampleTime=-1  HasFrameUpgradeWarning=on
  Tref : Outport
  wires:
  "Nm "/1 -> Sum/2
  ref_Speed/1 -> Sum/1
  Discrete-Time Integrator/1 -> Sum2/1
  Kp/1 -> Sum2/2
  KI/1 -> Discrete-Time Integrator/1
  Sum2/1 -> Saturation2/1, Unit Delay/1
  Saturation2/1 -> Tref/1, Unit Delay1/1
  Sign/1 -> Equal1/2
  Sign1/1 -> Equal1/1
  Equal1/1 -> AND/1
  Equal/1 -> AND/2
  Unit Delay/1 -> Equal/1, Sign/1
  Product/1 -> KI/1
  Unit Delay1/1 -> Equal/2
  AND/1 -> Product/1
  Sum/1 -> Kp/1, Sign1/1, Product/2

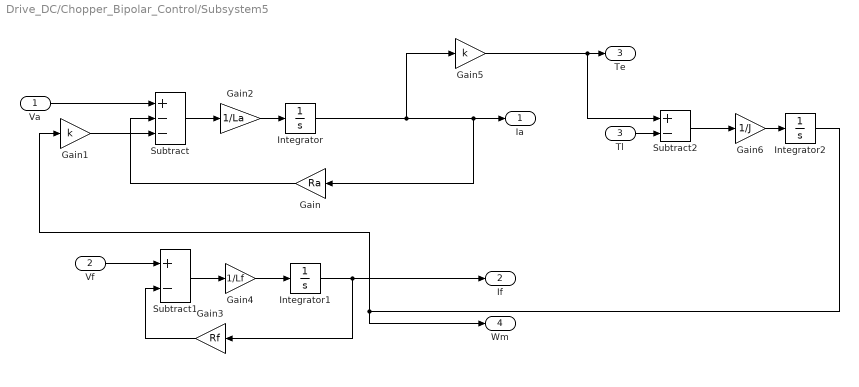
== system Drive_DC/Chopper_Bipolar_Control/Subsystem5 ==
  Va : Inport
  Vf : Inport  Port=2
  Tl : Inport  Port=3
  Gain : Gain  Gain=Ra
  Gain1 : Gain  Gain=k
  Gain2 : Gain  Gain=1/La
  Gain3 : Gain  Gain=Rf
  Gain4 : Gain  Gain=1/Lf
  Gain5 : Gain  Gain=k
  Gain6 : Gain  Gain=1/J
  Integrator : Integrator
  Integrator1 : Integrator
  Integrator2 : Integrator
  Subtract : Sum  Inputs=+--
  Subtract1 : Sum  Inputs=+-
  Subtract2 : Sum  Inputs=+-
  Ia : Outport
  If : Outport  Port=2
  Te : Outport  Port=3
  Wm : Outport  Port=4
  wires:
  Gain6/1 -> Integrator2/1
  Subtract2/1 -> Gain6/1
  Tl/1 -> Subtract2/2
  Gain5/1 -> Te/1, Subtract2/1
  Gain3/1 -> Subtract1/2
  Integrator1/1 -> If/1, Gain3/1
  Subtract1/1 -> Gain4/1
  Gain4/1 -> Integrator1/1
  Vf/1 -> Subtract1/1
  Gain2/1 -> Integrator/1
  Subtract/1 -> Gain2/1
  Gain1/1 -> Subtract/3
  Integrator2/1 -> Gain1/1, Wm/1
  Gain/1 -> Subtract/2
  Va/1 -> Subtract/1
  Integrator/1 -> Gain/1, Ia/1, Gain5/1

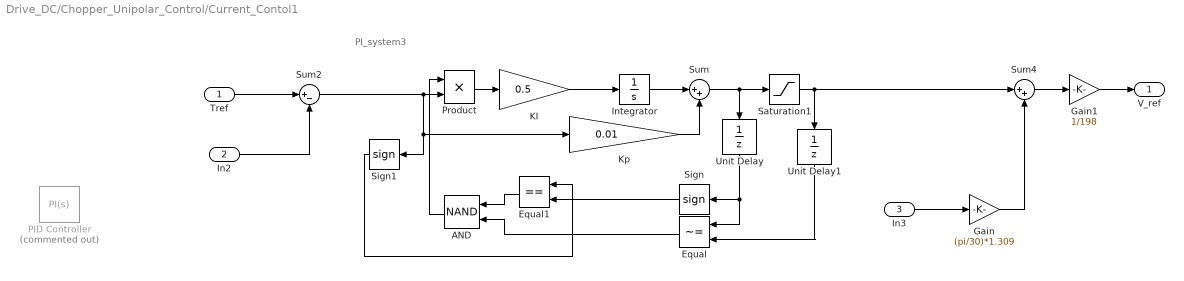
== system Drive_DC/Chopper_Unipolar_Control/Current_Contol1 ==
  note: PI_system3
  Tref : Inport
  In2 : Inport  Port=2
  In3 : Inport  Port=3
  AND : Logic  Operator=NAND  AllPortsSameDT=off  OutDataTypeStr=boolean
  Equal : RelationalOperator  Operator=~=  OutDataTypeStr=boolean  RndMeth=Simplest  InputSameDT=off
  Equal1 : RelationalOperator  Operator===  OutDataTypeStr=boolean  RndMeth=Simplest  InputSameDT=off
  Gain : Gain  Gain=(pi/30)*1.309
  Gain1 : Gain  Gain=1/198
  Integrator : Integrator
  KI : Gain  Gain=0.5
  Kp : Gain  Gain=0.01
  PID Controller : slpidlib/PID Controller  Commented=on  Controller=PI  Form=Parallel  TimeDomain=Continuous-time  UseExternalTs=off  SampleTime=-1  IntegratorMethod=Forward Euler  FilterMethod=Forward Euler  ControllerParametersSource=internal  P=0.1  I=10  UseKiTs=off  D=0  N=100  UseFilter=on  TunerSelectOption=Transfer Function Based (PID Tuner App)  InitialConditionSource=internal  InitialConditionForIntegrator=0  InitialConditionForFilter=0  DifferentiatorICPrevScaledInput=0  ExternalReset=none  TrackingMode=off  Kt=1  LimitOutput=on  SatLimitsSource=internal  UpperSaturationLimit=240  LowerSaturationLimit=-240  LinearizeAsGain=on  AntiWindupMode=clamping  Kb=1  LimitIntegrator=off  UpperIntegratorSaturationLimit=inf  LowerIntegratorSaturationLimit=-inf  POutMin=[]  POutMax=[]  IOutMin=[]  IOutMax=[]  DOutMin=[]  DOutMax=[]  NOutMin=[]  NOutMax=[]  SumOutMin=[]  SumOutMax=[]  SaturationOutMin=[]  SaturationOutMax=[]  PParamMin=[]  PParamMax=[]  IParamMin=[]  IParamMax=[]  DParamMin=[]  DParamMax=[]  NParamMin=[]  NParamMax=[]  KbParamMin=[]  KbParamMax=[]  KtParamMin=[]  KtParamMax=[]  KbOutMin=[]  KbOutMax=[]  KtOutMin=[]  KtOutMax=[]  IntegratorOutMin=[]  IntegratorOutMax=[]  FilterOutMin=[]  FilterOutMax=[]  SumI1OutMin=[]  SumI1OutMax=[]  SumI2OutMin=[]  SumI2OutMax=[]  SumI3OutMin=[]  SumI3OutMax=[]  SumI4OutMin=[]  SumI4OutMax=[]  SumDOutMin=[]  SumDOutMax=[]  DifferentiatorOutMin=[]  DifferentiatorOutMax=[]  FilterDiffOutCoefMin=[]  FilterDiffOutCoefMax=[]  ReciprocalOutMin=[]  ReciprocalOutMax=[]  SumDenOutMin=[]  SumDenOutMax=[]  SumNumOutMin=[]  SumNumOutMax=[]  DivideOutMin=[]  DivideOutMax=[]  UdiffTsProdOutMin=[]  UdiffTsProdOutMax=[]  NTsProdOutMin=[]  NTsProdOutMax=[]  UintegralTsProdOutMin=[]  UintegralTsProdOutMax=[]  UngainTsProdOutMin=[]  UngainTsProdOutMax=[]  ClampingZeroOutDataTypeStr=Inherit: Inherit via back propagation  ClampingZeroOutMin=[]  ClampingZeroOutMax=[]  FilterDenConstantOutDataTypeStr=Inherit: Inherit via back propagation  FilterDenConstantOutMin=[]  FilterDenConstantOutMax=[]  PCopyOutDataTypeStr=Inherit: Inherit via back propagation  PCopyOutMin=[]  PCopyOutMax=[]  NCopyOutDataTypeStr=Inherit: Inherit via back propagation  NCopyOutMin=[]  NCopyOutMax=[]  IntegratorContinuousStateAttributes=''  IntegratorStateMustResolveToSignalObject=off  IntegratorRTWStateStorageClass=Auto  FilterContinuousStateAttributes=''  FilterStateMustResolveToSignalObject=off  FilterRTWStateStorageClass=Auto  ParallelPVariant=InternalParameters  IdealPVariant=Disabled  IVariant=InternalParameters  DVariant=Disabled  IntegratorVariant=Continuous  SatVariant=Enabled  AWVariant=ContClampingParallel  PCopyVariant=Disabled  TRVariant=Disabled  FdbkBlocksVariant=Forward  IdealPFdbkVariant=Disabled  SatFdbkVariant=Disabled  DerivativeFilterVariant=Disabled  NVariant=Disabled  NCopyVariant=Disabled_SignalSpec  FilterICVariant=Disabled  IntegratorICVariant=InternalICs  ExternalResetVariant=Disabled  TRSumVariant=Passthrough  SumFdbkVariant=Disabled  SumVariant=Sum_PI  TsampFilterVariant=InternalTs  TsampNgainVariant=Passthrough  TsampIntegralVariant=Passthrough  ExternalSaturationOutDataTypeStr=Inherit: Same as second input
  Product : Product
  Saturation1 : Saturate  UpperLimit=198  LowerLimit=-198
  Sign : Signum
  Sign1 : Signum
  Sum : Sum  Inputs=|++
  Sum2 : Sum  Inputs=|+-
  Sum4 : Sum  Inputs=|++
  Unit Delay : UnitDelay  SampleTime=-1  HasFrameUpgradeWarning=on
  Unit Delay1 : UnitDelay  SampleTime=-1  HasFrameUpgradeWarning=on
  V_ref : Outport
  wires:
  Sum4/1 -> Gain1/1
  Sum2/1 -> Product/2, Sign1/1, Kp/1
  AND/1 -> Product/1
  Unit Delay1/1 -> Equal/2
  Product/1 -> KI/1
  Unit Delay/1 -> Sign/1, Equal/1
  Equal/1 -> AND/2
  Equal1/1 -> AND/1
  Sign1/1 -> Equal1/1
  Sign/1 -> Equal1/2
  Saturation1/1 -> Unit Delay1/1, Sum4/1
  Sum/1 -> Unit Delay/1, Saturation1/1
  KI/1 -> Integrator/1
  Kp/1 -> Sum/2
  Integrator/1 -> Sum/1
  Gain/1 -> Sum4/2
  In3/1 -> Gain/1
  In2/1 -> Sum2/2
  Tref/1 -> Sum2/1
  Gain1/1 -> V_ref/1

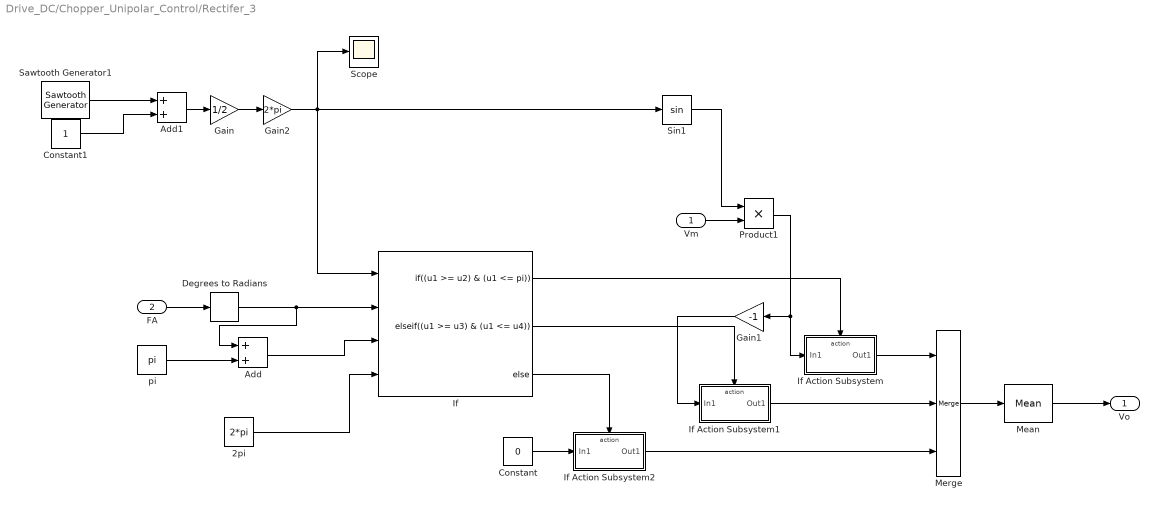
== system Drive_DC/Chopper_Unipolar_Control/Rectifer_3 ==
  Vm : Inport
  FA : Inport  Port=2
  2pi : Constant  Value=2*pi
  Add : Sum
  Add1 : Sum
  Constant : Constant  Value=0
  Constant1 : Constant
  Degrees to Radians : simulink_extras/Transformations/Degrees to Radians
  Gain : Gain  Gain=1/2
  Gain1 : Gain  Gain=-1
  Gain2 : Gain  Gain=2*pi
  If : If  NumInputs=4  IfExpression=(u1 >= u2) & (u1 <= pi)  ElseIfExpressions=(u1 >= u3) & (u1 <= u4)
  If Action Subsystem : Subsystem  TreatAsAtomicUnit=on
  If Action Subsystem1 : Subsystem  TreatAsAtomicUnit=on
  If Action Subsystem2 : Subsystem  TreatAsAtomicUnit=on
  Mean : spsMeanLib/Mean  Freq=50  Vinit=0  Ts=0
  Merge : Merge  Inputs=3
  Product1 : Product
  Sawtooth Generator1 : spsSawtoothGeneratorLib/Sawtooth Generator  Freq=50  Phase=180  Ts=0
  Scope : Scope
  Sin1 : Trigonometry
  pi : Constant  Value=pi
  Vo : Outport
  wires:
  Gain2/1 -> Sin1/1, If/1, Scope/1
  Gain/1 -> Gain2/1
  Add1/1 -> Gain/1
  Constant1/1 -> Add1/2
  Sawtooth Generator1/1 -> Add1/1
  Constant/1 -> If Action Subsystem2/1(In1)
  Gain1/1 -> If Action Subsystem1/1(In1)
  Product1/1 -> Gain1/1, If Action Subsystem/1(In1)
  Sin1/1 -> Product1/1
  Merge/1 -> Mean/1
  If Action Subsystem2/1(Out1) -> Merge/3
  If Action Subsystem1/1(Out1) -> Merge/2
  If Action Subsystem/1(Out1) -> Merge/1
  If/3 -> If Action Subsystem2/Action
  If/2 -> If Action Subsystem1/Action
  If/1 -> If Action Subsystem/Action
  2pi/1 -> If/4
  Add/1 -> If/3
  pi/1 -> Add/2
  Degrees to Radians/1 -> If/2, Add/1
  FA/1 -> Degrees to Radians/1
  Mean/1 -> Vo/1
  Vm/1 -> Product1/2

== system Drive_DC/Chopper_Unipolar_Control/Signal Builder1 ==
  Demux : Demux  Tag=STV Demux  Outputs=1
      settings: DisplayOption=none
  FromWs : FromWorkspace  Tag=STV FromWs  VariableName=tuvar
      SigBuilderData=|
      | common.afterFinalStr = 'Extrapolate'
      | common.sampleTime = 0
      | dataSet.timeRange = [0 13]
      | dataSet.name = 'Group 1'
      | sbobj.Groups.Name = 'Group 1'
      | sbobj.Groups.Signals.Name = 'Signal 1'
      | sbobj.Groups.Signals.XData = [0 1 2 3 4 5 8 9 10 11 12 13]
      | sbobj.Groups.Signals.YData = [0 0 0.5 0.5 1 1 -0.5 -0.5 -0.85 -0.85 -0.01 -0.01]
      | sbobj.Groups.TimeRange = [0 13]
  Signal 1 : Outport  Tag=STV Outport
  wires:
  FromWs/1 -> Demux/1
  Demux/1 -> Signal 1/1

== system Drive_DC/Chopper_Unipolar_Control/Speed_Control ==
  note: PI_system3
  In1 : Inport
  In2 : Inport  Port=2
  AND : Logic  Operator=NAND  AllPortsSameDT=off  OutDataTypeStr=boolean
  Equal : RelationalOperator  Operator=~=  OutDataTypeStr=boolean  RndMeth=Simplest  InputSameDT=off
  Equal1 : RelationalOperator  Operator===  OutDataTypeStr=boolean  RndMeth=Simplest  InputSameDT=off
  Integrator : Integrator
  KI : Gain  Gain=0.7
  Kp : Gain  Gain=0.5
  PID Controller : slpidlib/PID Controller  Commented=on  Controller=PI  Form=Parallel  TimeDomain=Continuous-time  UseExternalTs=off  SampleTime=-1  IntegratorMethod=Forward Euler  FilterMethod=Forward Euler  ControllerParametersSource=internal  P=0.5  I=0.5  UseKiTs=off  D=0  N=100  UseFilter=on  TunerSelectOption=Transfer Function Based (PID Tuner App)  InitialConditionSource=internal  InitialConditionForIntegrator=0  InitialConditionForFilter=0  DifferentiatorICPrevScaledInput=0  ExternalReset=none  TrackingMode=off  Kt=1  LimitOutput=on  SatLimitsSource=internal  UpperSaturationLimit=(30*746)/(1740*pi/30)  LowerSaturationLimit=-(30*746)/(1740*pi/30)  LinearizeAsGain=on  AntiWindupMode=clamping  Kb=1  LimitIntegrator=off  UpperIntegratorSaturationLimit=inf  LowerIntegratorSaturationLimit=-inf  POutMin=[]  POutMax=[]  IOutMin=[]  IOutMax=[]  DOutMin=[]  DOutMax=[]  NOutMin=[]  NOutMax=[]  SumOutMin=[]  SumOutMax=[]  SaturationOutMin=[]  SaturationOutMax=[]  PParamMin=[]  PParamMax=[]  IParamMin=[]  IParamMax=[]  DParamMin=[]  DParamMax=[]  NParamMin=[]  NParamMax=[]  KbParamMin=[]  KbParamMax=[]  KtParamMin=[]  KtParamMax=[]  KbOutMin=[]  KbOutMax=[]  KtOutMin=[]  KtOutMax=[]  IntegratorOutMin=[]  IntegratorOutMax=[]  FilterOutMin=[]  FilterOutMax=[]  SumI1OutMin=[]  SumI1OutMax=[]  SumI2OutMin=[]  SumI2OutMax=[]  SumI3OutMin=[]  SumI3OutMax=[]  SumI4OutMin=[]  SumI4OutMax=[]  SumDOutMin=[]  SumDOutMax=[]  DifferentiatorOutMin=[]  DifferentiatorOutMax=[]  FilterDiffOutCoefMin=[]  FilterDiffOutCoefMax=[]  ReciprocalOutMin=[]  ReciprocalOutMax=[]  SumDenOutMin=[]  SumDenOutMax=[]  SumNumOutMin=[]  SumNumOutMax=[]  DivideOutMin=[]  DivideOutMax=[]  UdiffTsProdOutMin=[]  UdiffTsProdOutMax=[]  NTsProdOutMin=[]  NTsProdOutMax=[]  UintegralTsProdOutMin=[]  UintegralTsProdOutMax=[]  UngainTsProdOutMin=[]  UngainTsProdOutMax=[]  ClampingZeroOutDataTypeStr=Inherit: Inherit via back propagation  ClampingZeroOutMin=[]  ClampingZeroOutMax=[]  FilterDenConstantOutDataTypeStr=Inherit: Inherit via back propagation  FilterDenConstantOutMin=[]  FilterDenConstantOutMax=[]  PCopyOutDataTypeStr=Inherit: Inherit via back propagation  PCopyOutMin=[]  PCopyOutMax=[]  NCopyOutDataTypeStr=Inherit: Inherit via back propagation  NCopyOutMin=[]  NCopyOutMax=[]  IntegratorContinuousStateAttributes=''  IntegratorStateMustResolveToSignalObject=off  IntegratorRTWStateStorageClass=Auto  FilterContinuousStateAttributes=''  FilterStateMustResolveToSignalObject=off  FilterRTWStateStorageClass=Auto  ParallelPVariant=InternalParameters  IdealPVariant=Disabled  IVariant=InternalParameters  DVariant=Disabled  IntegratorVariant=Continuous  SatVariant=Enabled  AWVariant=ContClampingParallel  PCopyVariant=Disabled  TRVariant=Disabled  FdbkBlocksVariant=Forward  IdealPFdbkVariant=Disabled  SatFdbkVariant=Disabled  DerivativeFilterVariant=Disabled  NVariant=Disabled  NCopyVariant=Disabled_SignalSpec  FilterICVariant=Disabled  IntegratorICVariant=InternalICs  ExternalResetVariant=Disabled  TRSumVariant=Passthrough  SumFdbkVariant=Disabled  SumVariant=Sum_PI  TsampFilterVariant=InternalTs  TsampNgainVariant=Passthrough  TsampIntegralVariant=Passthrough  ExternalSaturationOutDataTypeStr=Inherit: Same as second input
  Product : Product
  Saturation1 : Saturate  UpperLimit=(30*746)/(1740*pi/30)  LowerLimit=-(30*746)/(1740*pi/30)
  Sign : Signum
  Sign1 : Signum
  Sum : Sum  Inputs=|+-
  Sum2 : Sum  Inputs=|++
  Unit Delay : UnitDelay  SampleTime=-1  HasFrameUpgradeWarning=on
  Unit Delay1 : UnitDelay  SampleTime=-1  HasFrameUpgradeWarning=on
  Tref : Outport
  wires:
  Sum/1 -> Product/2, Sign1/1, Kp/1
  AND/1 -> Product/1
  Unit Delay1/1 -> Equal/2
  Product/1 -> KI/1
  Unit Delay/1 -> Sign/1, Equal/1
  Equal/1 -> AND/2
  Equal1/1 -> AND/1
  Sign1/1 -> Equal1/1
  Sign/1 -> Equal1/2
  Saturation1/1 -> Unit Delay1/1, Tref/1
  Sum2/1 -> Unit Delay/1, Saturation1/1
  KI/1 -> Integrator/1
  Kp/1 -> Sum2/2
  Integrator/1 -> Sum2/1
  In1/1 -> Sum/1
  In2/1 -> Sum/2

== system Drive_DC/Chopper_Unipolar_Control/Subsystem5 ==
  Va : Inport
  Vf : Inport  Port=2
  Tl : Inport  Port=3
  Gain : Gain  Gain=Ra
  Gain1 : Gain  Gain=k
  Gain2 : Gain  Gain=1/La
  Gain3 : Gain  Gain=Rf
  Gain4 : Gain  Gain=1/Lf
  Gain5 : Gain  Gain=k
  Gain6 : Gain  Gain=1/J
  Integrator : Integrator
  Integrator1 : Integrator
  Integrator2 : Integrator
  Subtract : Sum  Inputs=+--
  Subtract1 : Sum  Inputs=+-
  Subtract2 : Sum  Inputs=+-
  Ia : Outport
  If : Outport  Port=2
  Te : Outport  Port=3
  Wm : Outport  Port=4
  wires:
  Integrator/1 -> Gain5/1, Ia/1, Gain/1
  Va/1 -> Subtract/1
  Gain/1 -> Subtract/2
  Integrator2/1 -> Wm/1, Gain1/1
  Gain1/1 -> Subtract/3
  Subtract/1 -> Gain2/1
  Gain2/1 -> Integrator/1
  Vf/1 -> Subtract1/1
  Gain4/1 -> Integrator1/1
  Subtract1/1 -> Gain4/1
  Integrator1/1 -> Gain3/1, If/1
  Gain3/1 -> Subtract1/2
  Gain5/1 -> Subtract2/1, Te/1
  Tl/1 -> Subtract2/2
  Subtract2/1 -> Gain6/1
  Gain6/1 -> Integrator2/1

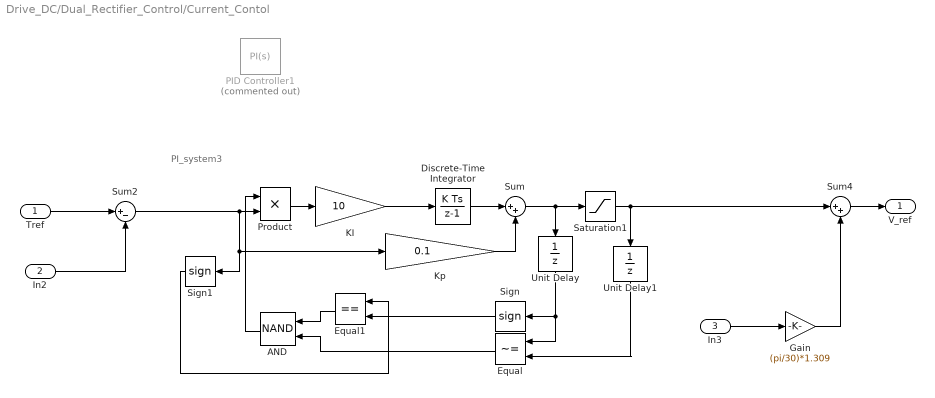
== system Drive_DC/Dual_Rectifier_Control/Current_Contol ==
  note: PI_system3
  Tref : Inport
  In2 : Inport  Port=2
  In3 : Inport  Port=3
  AND : Logic  Operator=NAND  AllPortsSameDT=off  OutDataTypeStr=boolean
  Discrete-Time Integrator : DiscreteIntegrator  SampleTime=-1  ICPrevOutput=DiscIntNeverNeededParam  ICPrevScaledInput=DiscIntNeverNeededParam
  Equal : RelationalOperator  Operator=~=  OutDataTypeStr=boolean  RndMeth=Simplest  InputSameDT=off
  Equal1 : RelationalOperator  Operator===  OutDataTypeStr=boolean  RndMeth=Simplest  InputSameDT=off
  Gain : Gain  Gain=(pi/30)*1.309
  KI : Gain  Gain=10
  Kp : Gain  Gain=0.1
  PID Controller1 : slpidlib/PID Controller  Commented=on  Controller=PI  Form=Parallel  TimeDomain=Continuous-time  UseExternalTs=off  SampleTime=-1  IntegratorMethod=Forward Euler  FilterMethod=Forward Euler  ControllerParametersSource=internal  P=0.1  I=10  UseKiTs=off  D=0  N=100  UseFilter=on  TunerSelectOption=Transfer Function Based (PID Tuner App)  InitialConditionSource=internal  InitialConditionForIntegrator=0  InitialConditionForFilter=0  DifferentiatorICPrevScaledInput=0  ExternalReset=none  TrackingMode=off  Kt=1  LimitOutput=on  SatLimitsSource=internal  UpperSaturationLimit=198  LowerSaturationLimit=-198  LinearizeAsGain=on  AntiWindupMode=clamping  Kb=1  LimitIntegrator=off  UpperIntegratorSaturationLimit=inf  LowerIntegratorSaturationLimit=-inf  POutMin=[]  POutMax=[]  IOutMin=[]  IOutMax=[]  DOutMin=[]  DOutMax=[]  NOutMin=[]  NOutMax=[]  SumOutMin=[]  SumOutMax=[]  SaturationOutMin=[]  SaturationOutMax=[]  PParamMin=[]  PParamMax=[]  IParamMin=[]  IParamMax=[]  DParamMin=[]  DParamMax=[]  NParamMin=[]  NParamMax=[]  KbParamMin=[]  KbParamMax=[]  KtParamMin=[]  KtParamMax=[]  KbOutMin=[]  KbOutMax=[]  KtOutMin=[]  KtOutMax=[]  IntegratorOutMin=[]  IntegratorOutMax=[]  FilterOutMin=[]  FilterOutMax=[]  SumI1OutMin=[]  SumI1OutMax=[]  SumI2OutMin=[]  SumI2OutMax=[]  SumI3OutMin=[]  SumI3OutMax=[]  SumI4OutMin=[]  SumI4OutMax=[]  SumDOutMin=[]  SumDOutMax=[]  DifferentiatorOutMin=[]  DifferentiatorOutMax=[]  FilterDiffOutCoefMin=[]  FilterDiffOutCoefMax=[]  ReciprocalOutMin=[]  ReciprocalOutMax=[]  SumDenOutMin=[]  SumDenOutMax=[]  SumNumOutMin=[]  SumNumOutMax=[]  DivideOutMin=[]  DivideOutMax=[]  UdiffTsProdOutMin=[]  UdiffTsProdOutMax=[]  NTsProdOutMin=[]  NTsProdOutMax=[]  UintegralTsProdOutMin=[]  UintegralTsProdOutMax=[]  UngainTsProdOutMin=[]  UngainTsProdOutMax=[]  ClampingZeroOutDataTypeStr=Inherit: Inherit via back propagation  ClampingZeroOutMin=[]  ClampingZeroOutMax=[]  FilterDenConstantOutDataTypeStr=Inherit: Inherit via back propagation  FilterDenConstantOutMin=[]  FilterDenConstantOutMax=[]  PCopyOutDataTypeStr=Inherit: Inherit via back propagation  PCopyOutMin=[]  PCopyOutMax=[]  NCopyOutDataTypeStr=Inherit: Inherit via back propagation  NCopyOutMin=[]  NCopyOutMax=[]  IntegratorContinuousStateAttributes=''  IntegratorStateMustResolveToSignalObject=off  IntegratorRTWStateStorageClass=Auto  FilterContinuousStateAttributes=''  FilterStateMustResolveToSignalObject=off  FilterRTWStateStorageClass=Auto  ParallelPVariant=InternalParameters  IdealPVariant=Disabled  IVariant=InternalParameters  DVariant=Disabled  IntegratorVariant=Continuous  SatVariant=Enabled  AWVariant=ContClampingParallel  PCopyVariant=Disabled  TRVariant=Disabled  FdbkBlocksVariant=Forward  IdealPFdbkVariant=Disabled  SatFdbkVariant=Disabled  DerivativeFilterVariant=Disabled  NVariant=Disabled  NCopyVariant=Disabled_SignalSpec  FilterICVariant=Disabled  IntegratorICVariant=InternalICs  ExternalResetVariant=Disabled  TRSumVariant=Passthrough  SumFdbkVariant=Disabled  SumVariant=Sum_PI  TsampFilterVariant=InternalTs  TsampNgainVariant=Passthrough  TsampIntegralVariant=Passthrough  ExternalSaturationOutDataTypeStr=Inherit: Same as second input
  Product : Product
  Saturation1 : Saturate  UpperLimit=198  LowerLimit=-198
  Sign : Signum
  Sign1 : Signum
  Sum : Sum  Inputs=|++
  Sum2 : Sum  Inputs=|+-
  Sum4 : Sum  Inputs=|++
  Unit Delay : UnitDelay  SampleTime=-1  HasFrameUpgradeWarning=on
  Unit Delay1 : UnitDelay  SampleTime=-1  HasFrameUpgradeWarning=on
  V_ref : Outport
  wires:
  Tref/1 -> Sum2/1
  In2/1 -> Sum2/2
  In3/1 -> Gain/1
  Gain/1 -> Sum4/2
  Discrete-Time Integrator/1 -> Sum/1
  Kp/1 -> Sum/2
  KI/1 -> Discrete-Time Integrator/1
  Sum/1 -> Saturation1/1, Unit Delay/1
  Saturation1/1 -> Sum4/1, Unit Delay1/1
  Sign/1 -> Equal1/2
  Sign1/1 -> Equal1/1
  Equal1/1 -> AND/1
  Equal/1 -> AND/2
  Unit Delay/1 -> Equal/1, Sign/1
  Product/1 -> KI/1
  Unit Delay1/1 -> Equal/2
  AND/1 -> Product/1
  Sum2/1 -> Kp/1, Sign1/1, Product/2
  Sum4/1 -> V_ref/1

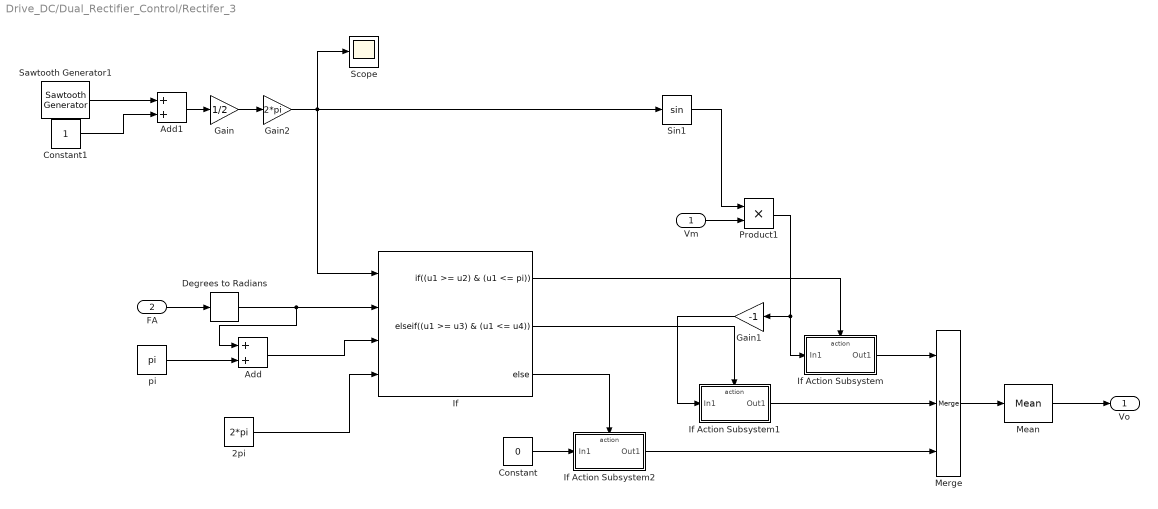
== system Drive_DC/Dual_Rectifier_Control/Rectifer_3 ==
  Vm : Inport
  FA : Inport  Port=2
  2pi : Constant  Value=2*pi
  Add : Sum
  Add1 : Sum
  Constant : Constant  Value=0
  Constant1 : Constant
  Degrees to Radians : simulink_extras/Transformations/Degrees to Radians
  Gain : Gain  Gain=1/2
  Gain1 : Gain  Gain=-1
  Gain2 : Gain  Gain=2*pi
  If : If  NumInputs=4  IfExpression=(u1 >= u2) & (u1 <= pi)  ElseIfExpressions=(u1 >= u3) & (u1 <= u4)
  If Action Subsystem : Subsystem  TreatAsAtomicUnit=on
  If Action Subsystem1 : Subsystem  TreatAsAtomicUnit=on
  If Action Subsystem2 : Subsystem  TreatAsAtomicUnit=on
  Mean : spsMeanLib/Mean  Freq=50  Vinit=0  Ts=0
  Merge : Merge  Inputs=3
  Product1 : Product
  Sawtooth Generator1 : spsSawtoothGeneratorLib/Sawtooth Generator  Freq=50  Phase=180  Ts=0
  Scope : Scope
  Sin1 : Trigonometry
  pi : Constant  Value=pi
  Vo : Outport
  wires:
  Gain2/1 -> Sin1/1, If/1, Scope/1
  Gain/1 -> Gain2/1
  Add1/1 -> Gain/1
  Constant1/1 -> Add1/2
  Sawtooth Generator1/1 -> Add1/1
  Constant/1 -> If Action Subsystem2/1(In1)
  Gain1/1 -> If Action Subsystem1/1(In1)
  Product1/1 -> Gain1/1, If Action Subsystem/1(In1)
  Sin1/1 -> Product1/1
  Merge/1 -> Mean/1
  If Action Subsystem2/1(Out1) -> Merge/3
  If Action Subsystem1/1(Out1) -> Merge/2
  If Action Subsystem/1(Out1) -> Merge/1
  If/3 -> If Action Subsystem2/Action
  If/2 -> If Action Subsystem1/Action
  If/1 -> If Action Subsystem/Action
  2pi/1 -> If/4
  Add/1 -> If/3
  pi/1 -> Add/2
  Degrees to Radians/1 -> If/2, Add/1
  FA/1 -> Degrees to Radians/1
  Mean/1 -> Vo/1
  Vm/1 -> Product1/2

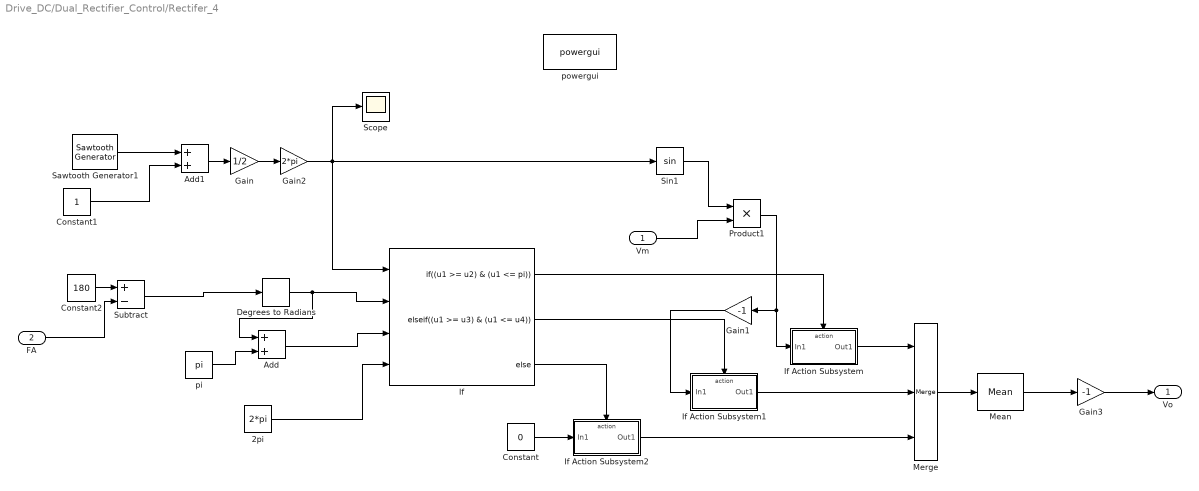
== system Drive_DC/Dual_Rectifier_Control/Rectifer_4 ==
  Vm : Inport
  FA : Inport  Port=2
  2pi : Constant  Value=2*pi
  Add : Sum
  Add1 : Sum
  Constant : Constant  Value=0
  Constant1 : Constant
  Constant2 : Constant  Value=180
  Degrees to Radians : simulink_extras/Transformations/Degrees to Radians
  Gain : Gain  Gain=1/2
  Gain1 : Gain  Gain=-1
  Gain2 : Gain  Gain=2*pi
  Gain3 : Gain  Gain=-1
  If : If  NumInputs=4  IfExpression=(u1 >= u2) & (u1 <= pi)  ElseIfExpressions=(u1 >= u3) & (u1 <= u4)
  If Action Subsystem : Subsystem  TreatAsAtomicUnit=on
  If Action Subsystem1 : Subsystem  TreatAsAtomicUnit=on
  If Action Subsystem2 : Subsystem  TreatAsAtomicUnit=on
  Mean : spsMeanLib/Mean  Freq=50  Vinit=0  Ts=0
  Merge : Merge  Inputs=3
  Product1 : Product
  Sawtooth Generator1 : spsSawtoothGeneratorLib/Sawtooth Generator  Freq=50  Phase=180  Ts=0
  Scope : Scope
  Sin1 : Trigonometry
  Subtract : Sum  Inputs=+-
  pi : Constant  Value=pi
  powergui : spspowerguiLib/powergui  Priority=1  SimulationMode=Continuous  SampleTime=50e-6  frequency=60  Iterations=50  frequencyindice=50  Pbase=100e6  ErrMax=1e-4  UnitsV=kV  UnitsW=MW  buscounter=0  FunctionMessages=off  echomessages=off  EnableUseOfTLC=off  CurrentSourceSwitches=off  DisableSnubberDevices=off  DisableRonSwitches=off  DisableVfSwitches=off  DisplayEquations=off  AutomaticDiscreteSolvers=off  SolverType=Tustin/Backward Euler (TBE)  Interpol=off  ExternalGateDelay=off  methode=off  Ts=100  x0status=blocks  SPID=on  SwTol=0  HookPort=off  NonlinearTolerance=1e-4  nMaxIteration=100  ContinueOnMaxIteration=off  RestoreLinks=warning  ResistiveCurrentMeasurement=off  Frange=[0:2:500]  Ylog=off  Xlog=on  ShowGrid=off  save=off  variable=ZData  structure=0  ZoomFFT=off  StartTime=0.0  cycles=1  DisplayStyle=1  fundamental=60  FreqAxis=off  MaxFrequency=1000  frequencyindicesteady=1  RmsSteady=1  display=off
  Vo : Outport
  wires:
  Gain3/1 -> Vo/1
  FA/1 -> Subtract/2
  Degrees to Radians/1 -> Add/1, If/2
  pi/1 -> Add/2
  Add/1 -> If/3
  2pi/1 -> If/4
  If/1 -> If Action Subsystem/Action
  If/2 -> If Action Subsystem1/Action
  If/3 -> If Action Subsystem2/Action
  If Action Subsystem/1(Out1) -> Merge/1
  If Action Subsystem1/1(Out1) -> Merge/2
  If Action Subsystem2/1(Out1) -> Merge/3
  Merge/1 -> Mean/1
  Sin1/1 -> Product1/1
  Vm/1 -> Product1/2
  Product1/1 -> If Action Subsystem/1(In1), Gain1/1
  Gain1/1 -> If Action Subsystem1/1(In1)
  Constant/1 -> If Action Subsystem2/1(In1)
  Sawtooth Generator1/1 -> Add1/1
  Constant1/1 -> Add1/2
  Add1/1 -> Gain/1
  Gain/1 -> Gain2/1
  Gain2/1 -> Scope/1, If/1, Sin1/1
  Mean/1 -> Gain3/1
  Constant2/1 -> Subtract/1
  Subtract/1 -> Degrees to Radians/1

== system Drive_DC/Dual_Rectifier_Control/Signal Builder1 ==
  Demux : Demux  Tag=STV Demux  Outputs=1
      settings: DisplayOption=none
  FromWs : FromWorkspace  Tag=STV FromWs  VariableName=tuvar
      SigBuilderData=|
      | common.afterFinalStr = 'Extrapolate'
      | common.sampleTime = 0
      | dataSet.timeRange = [0 13]
      | dataSet.name = 'Group 1'
      | sbobj.Groups.Name = 'Group 1'
      | sbobj.Groups.Signals.Name = 'Signal 1'
      | sbobj.Groups.Signals.XData = [0 1 2 3 4 5 8 9 10 11 12 13]
      | sbobj.Groups.Signals.YData = [0 0 0.5 0.5 1 1 -0.5 -0.5 -0.85 -0.85 -0.01 -0.01]
      | sbobj.Groups.TimeRange = [0 13]
  Signal 1 : Outport  Tag=STV Outport
  wires:
  Demux/1 -> Signal 1/1
  FromWs/1 -> Demux/1
